simulink model "GHAME_Public"  (R2024a)
settings: Solver=ode8  StartTime=0.0  StopTime=Sim.simulation.duration  FixedStep=0.01  RelTol=1e-3
undefined symbols (not defined in the file): Data, DataPlant, IC, Sim, v0_BE_B
libraries: simulink_extras x8, simulink x1
(part 1 of 3)
settings Model: PacingRate=1000  Creator=Thoma  LastModifiedBy=muel_td
settings SolverCC: AlgebraicLoopSolver=TrustRegion  PositivePriorityOrder=on  MinimalZcImpactIntegration=on
settings DataIOCC: ExternalInput=getinputstruct(report2)  InitialState=getstatestruct(report2)
settings OptimizationCC: SimCompilerOptimization=on  AccelVerboseBuild=on
settings DebuggingCC: RTPrefix=none  StringTruncationChecking=none  ReadBeforeWriteMsg=DisableAll  WriteAfterWriteMsg=DisableAll  WriteAfterReadMsg=DisableAll  AlgebraicLoopMsg=none  SignalResolutionControl=None  MultiTaskDSMMsg=none  IntegerOverflowMsg=none  ParameterDowncastMsg=none  ParameterOverflowMsg=none  ParameterPrecisionLossMsg=none  ParameterTunabilityLossMsg=none  IntegerSaturationMsg=none  ArithmeticOperatorsInVariantConditions=warning
settings ModelReferenceCC: UpdateModelReferenceTargets=IfOutOfDate
settings SFSimCC: SFSimEcho=off  CustomCodeUndefinedFunction=UseInterfaceOnly
settings RTWCC: GPUComputeCapability=3.5

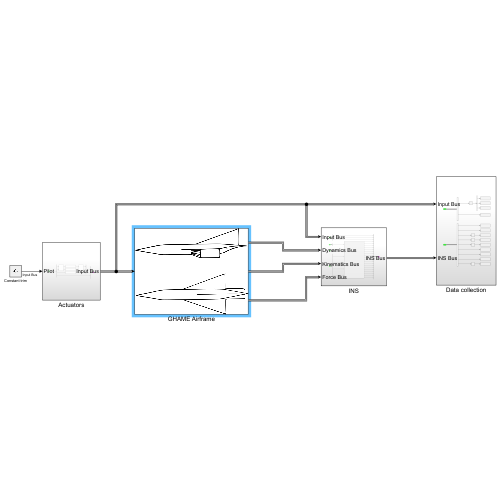
[thumbnail: Simulink's stored preview of the top-level diagram]
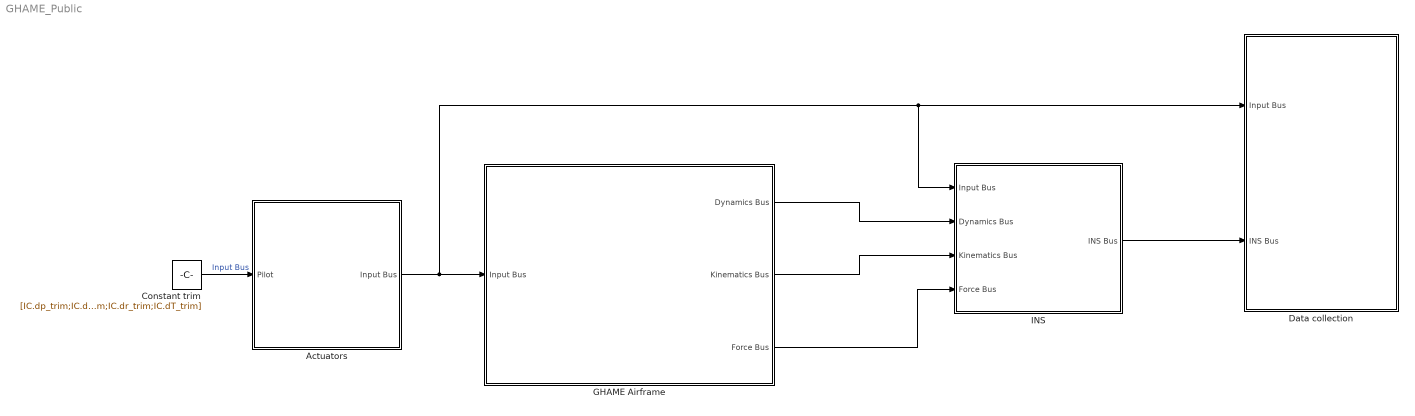
== system GHAME_Public ==
  Actuators : Subsystem
  Constant trim : Constant  Value=[IC.dp_trim;IC.dq_trim;IC.dr_trim;IC.dT_trim]
  Data collection : Subsystem
  GHAME Airframe : Subsystem
      mask Display: image('GHAME.png');
  INS : Subsystem
  wires:
  Actuators/1(Input Bus) -> GHAME Airframe/1(Input Bus), INS/1(Input Bus), Data collection/1(Input Bus)
  Constant trim/1 -> Actuators/1(Pilot)  "Input Bus"
  GHAME Airframe/2(Kinematics Bus) -> INS/3(Kinematics Bus)
  GHAME Airframe/1(Dynamics Bus) -> INS/2(Dynamics Bus)
  INS/1(INS Bus) -> Data collection/2(INS Bus)
  GHAME Airframe/3(Force Bus) -> INS/4(Force Bus)

== system GHAME_Public/Actuators ==
  Pilot : Inport
  Bus Creator : BusCreator  Inputs=2
  Demux : Demux
  Mux : Mux  Inputs=3
  Subsystem : Subsystem
  Subsystem1 : Subsystem
  Subsystem2 : Subsystem
  from Elevon command : Subsystem
  to Elevon command : Subsystem
  Input Bus : Outport
  wires:
  from Elevon command/1(dela) -> Mux/1  "Aileron"
  Demux/3 -> Subsystem2/1(delrc)
  to Elevon command/2(elvrc) -> Subsystem1/1(elvrc)
  Demux/1 -> to Elevon command/1(delac)
  to Elevon command/1(elvlc) -> Subsystem/1(elvlc)
  Demux/2 -> to Elevon command/2(delec)
  Subsystem/1(elvl) -> from Elevon command/1(elvl)
  Subsystem2/1(delr) -> Mux/3  "Rudder"
  Bus Creator/1 -> Input Bus/1
  Demux/4 -> Bus Creator/2  "thrtl"
  from Elevon command/2(dele) -> Mux/2  "Elevator"
  Mux/1 -> Bus Creator/1  "Deflections (rad)"
  Subsystem1/1(elvr) -> from Elevon command/2(elvr)
  Pilot/1 -> Demux/1

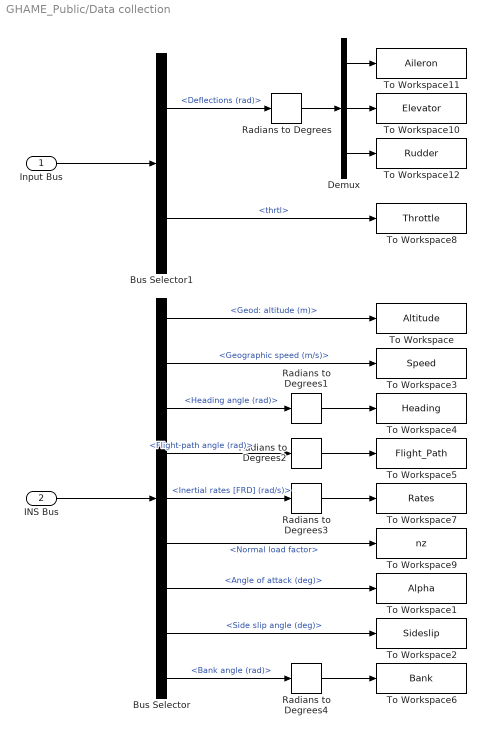
== system GHAME_Public/Data collection ==
  Input Bus : Inport
  INS Bus : Inport  Port=2
  Bus Selector : BusSelector  OutputSignals=Geod: altitude (m),Geographic speed (m/s),Heading angle (rad),Flight-path angle (rad),Inertial rates [FRD] (rad/s),Normal load factor,Angle of attack (deg),Side slip angle (deg),Bank angle (rad)
  Bus Selector1 : BusSelector  OutputSignals=Deflections (rad),thrtl
  Demux : Demux  Outputs=3
  Radians to Degrees{,1..4} (5 alike) : simulink_extras/Transformations/Radians to Degrees
  To Workspace : ToWorkspace  VariableName=Altitude  SampleTime=Sim.sample_time
  To Workspace1 : ToWorkspace  VariableName=Alpha  SampleTime=Sim.sample_time
  To Workspace10 : ToWorkspace  VariableName=Elevator  SampleTime=Sim.sample_time
  To Workspace11 : ToWorkspace  VariableName=Aileron  SampleTime=Sim.sample_time
  To Workspace12 : ToWorkspace  VariableName=Rudder  SampleTime=Sim.sample_time
  To Workspace2 : ToWorkspace  VariableName=Sideslip  SampleTime=Sim.sample_time
  To Workspace3 : ToWorkspace  VariableName=Speed  SampleTime=Sim.sample_time
  To Workspace4 : ToWorkspace  VariableName=Heading  SampleTime=Sim.sample_time
  To Workspace5 : ToWorkspace  VariableName=Flight_Path  SampleTime=Sim.sample_time
  To Workspace6 : ToWorkspace  VariableName=Bank  SampleTime=Sim.sample_time
  To Workspace7 : ToWorkspace  VariableName=Rates  SampleTime=Sim.sample_time
  To Workspace8 : ToWorkspace  VariableName=Throttle  SampleTime=Sim.sample_time
  To Workspace9 : ToWorkspace  VariableName=nz  SampleTime=Sim.sample_time
  wires:
  INS Bus/1 -> Bus Selector/1
  Bus Selector/1 -> To Workspace/1  "<Geod: altitude (m)>"
  Bus Selector/2 -> To Workspace3/1  "<Geographic speed (m/s)>"
  Bus Selector/3 -> Radians to Degrees1/1  "<Heading angle (rad)>"
  Bus Selector/4 -> Radians to Degrees2/1  "<Flight-path angle (rad)>"
  Bus Selector/5 -> Radians to Degrees3/1  "<Inertial rates [FRD] (rad/s)>"
  Bus Selector/6 -> To Workspace9/1  "<Normal load factor>"
  Bus Selector/7 -> To Workspace1/1  "<Angle of attack (deg)>"
  Bus Selector/8 -> To Workspace2/1  "<Side slip angle (deg)>"
  Bus Selector/9 -> Radians to Degrees4/1  "<Bank angle (rad)>"
  Input Bus/1 -> Bus Selector1/1
  Demux/1 -> To Workspace11/1
  Demux/2 -> To Workspace10/1
  Demux/3 -> To Workspace12/1
  Radians to Degrees1/1 -> To Workspace4/1
  Radians to Degrees2/1 -> To Workspace5/1
  Radians to Degrees3/1 -> To Workspace7/1
  Radians to Degrees4/1 -> To Workspace6/1
  Radians to Degrees/1 -> Demux/1
  Bus Selector1/2 -> To Workspace8/1  "<thrtl>"
  Bus Selector1/1 -> Radians to Degrees/1  "<Deflections (rad)>"

== system GHAME_Public/GHAME Airframe ==
  Input Bus : Inport
  Dynamics : Subsystem  Priority=4
  Environment : Subsystem  Priority=1
  Forces and Moments : Subsystem
  Kinematics : Subsystem  Priority=2
  Dynamics Bus : Outport
  Kinematics Bus : Outport  Port=2
  Force Bus : Outport  Port=3
  wires:
  Kinematics/1(Kinematics Bus) -> Forces and Moments/4(Kinematics Bus), Environment/2(Kinematics Bus), Kinematics Bus/1, Dynamics/3(Kinematics Bus)
  Dynamics/1(Dynamics Bus) -> Dynamics Bus/1, Forces and Moments/2(Dynamics Bus), Environment/1(Dynamics Bus), Kinematics/1(Dynamics Bus)
  Environment/1(Environment Bus) -> Forces and Moments/3(Environment Bus), Dynamics/2(Environment Bus)
  Forces and Moments/1(Force Bus) -> Dynamics/1(Force Bus), Force Bus/1
  Input Bus/1 -> Forces and Moments/1(Input Bus)

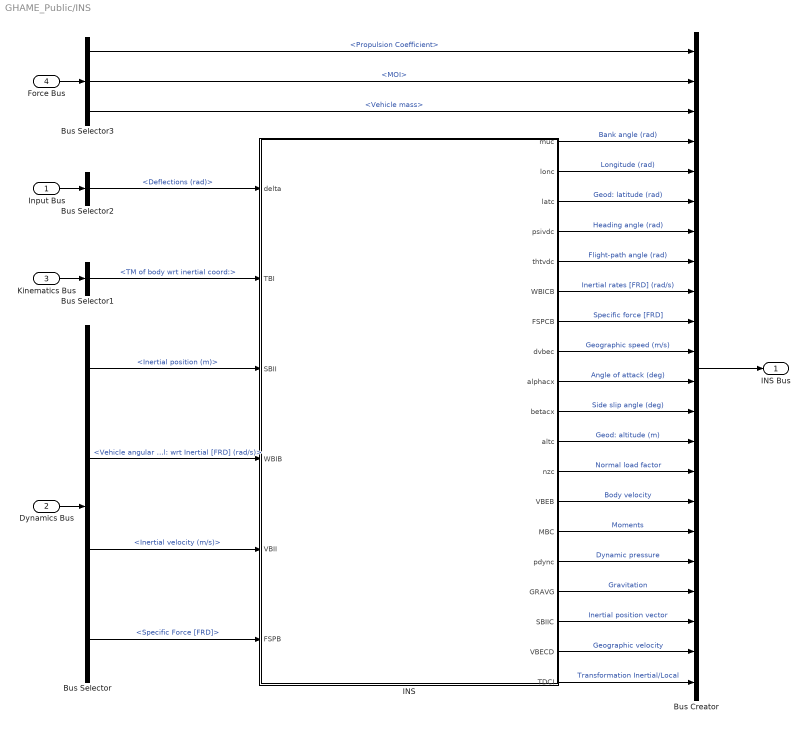
== system GHAME_Public/INS ==
  Input Bus : Inport
  Dynamics Bus : Inport  Port=2
  Kinematics Bus : Inport  Port=3
  Force Bus : Inport  Port=4
  Bus Creator : BusCreator  Inputs=22
  Bus Selector : BusSelector  OutputSignals=Newton Bus.Inertial position (m),Euler Bus.Vehicle angular vel: wrt Inertial [FRD] (rad/s),Newton Bus.Inertial velocity (m/s),Newton Bus.Specific Force [FRD]
  Bus Selector1 : BusSelector  OutputSignals=TM of body wrt inertial coord:
  Bus Selector2 : BusSelector  OutputSignals=Deflections (rad)
  Bus Selector3 : BusSelector  OutputSignals=Prop: data.Propulsion Coefficient,Prop: data.Mass and MOI.MOI,Prop: data.Mass and MOI.Vehicle mass
  INS : Subsystem
  INS Bus : Outport
  wires:
  INS/7(FSPCB) -> Bus Creator/10  "Specific force [FRD]"
  INS/5(thtvdc) -> Bus Creator/8  "Flight-path angle (rad)"
  INS/8(dvbec) -> Bus Creator/11  "Geographic speed (m/s)"
  INS/9(alphacx) -> Bus Creator/12  "Angle of attack (deg)"
  INS/6(WBICB) -> Bus Creator/9  "Inertial rates [FRD] (rad/s)"
  INS/4(psivdc) -> Bus Creator/7  "Heading angle (rad)"
  INS/10(betacx) -> Bus Creator/13  "Side slip angle (deg)"
  INS/1(muc) -> Bus Creator/4  "Bank angle (rad)"
  INS/2(lonc) -> Bus Creator/5  "Longitude (rad)"
  INS/11(altc) -> Bus Creator/14  "Geod: altitude (m)"
  INS/3(latc) -> Bus Creator/6  "Geod: latitude (rad)"
  Bus Selector/1 -> INS/3(SBII)  "<Inertial position (m)>"
  Bus Selector/3 -> INS/5(VBII)  "<Inertial velocity (m/s)>"
  Dynamics Bus/1 -> Bus Selector/1
  Bus Selector/2 -> INS/4(WBIB)  "<Vehicle angular vel: wrt Inertial [FRD] (rad/s)>"
  Bus Selector/4 -> INS/6(FSPB)  "<Specific Force [FRD]>"
  Kinematics Bus/1 -> Bus Selector1/1
  Bus Selector1/1 -> INS/2(TBI)  "<TM of body wrt inertial coord:>"
  Bus Creator/1 -> INS Bus/1
  INS/12(nzc) -> Bus Creator/15  "Normal load factor"
  INS/13(VBEB) -> Bus Creator/16  "Body velocity"
  Input Bus/1 -> Bus Selector2/1
  Bus Selector2/1 -> INS/1(delta)  "<Deflections (rad)>"
  Force Bus/1 -> Bus Selector3/1
  Bus Selector3/2 -> Bus Creator/2  "<MOI>"
  INS/14(MBC) -> Bus Creator/17  "Moments"
  INS/15(pdync) -> Bus Creator/18  "Dynamic pressure"
  Bus Selector3/3 -> Bus Creator/3  "<Vehicle mass>"
  INS/16(GRAVG) -> Bus Creator/19  "Gravitation"
  Bus Selector3/1 -> Bus Creator/1  "<Propulsion Coefficient>"
  INS/17(SBIIC) -> Bus Creator/20  "Inertial position vector"
  INS/18(VBECD) -> Bus Creator/21  "Geographic velocity"
  INS/19(TDCI) -> Bus Creator/22  "Transformation Inertial/Local"

== system GHAME_Public/Actuators/Subsystem ==
  elvlc : Inport
  2*zeta * wn : Gain  Gain=2*Sim.actuator.zeta*Sim.actuator.omega  SaturateOnIntegerOverflow=on  OutDataTypeStr=Inherit: Same as input  ParamDataTypeStr=Inherit: Same as input
  Demand limits : Saturate  UpperLimit=Sim.actuator.defl_lim_deg*Sim.constants.RAD  LowerLimit=-Sim.actuator.defl_lim_deg*Sim.constants.RAD
  "Integrator, Second-Order Limited" : SecondOrderIntegrator  ICX=IC.dp_trim+IC.dq_trim  LimitX=on  UpperLimitX=Sim.actuator.defl_lim_deg*Sim.constants.RAD  LowerLimitX=-Sim.actuator.defl_lim_deg*Sim.constants.RAD  ICDXDT=0  LimitDXDT=on  UpperLimitDXDT=Sim.actuator.rate_lim_deg*Sim.constants.RAD  LowerLimitDXDT=-Sim.actuator.rate_lim_deg*Sim.constants.RAD
  Sum2 : Sum  Inputs=|+-  InputSameDT=on  SaturateOnIntegerOverflow=on  OutDataTypeStr=Inherit: Same as first input
  Sum3 : Sum  Inputs=|+-  InputSameDT=on  SaturateOnIntegerOverflow=on  OutDataTypeStr=Inherit: Same as first input
  rate limit*2*zeta/wn : Saturate  UpperLimit=Sim.actuator.rate_lim_deg*2*Sim.actuator.zeta/Sim.actuator.omega*Sim.constants.RAD  LowerLimit=-Sim.actuator.rate_lim_deg*2*Sim.actuator.zeta/Sim.actuator.omega*Sim.constants.RAD
  wn^2 : Gain  Gain=Sim.actuator.omega^2  SaturateOnIntegerOverflow=on  OutDataTypeStr=Inherit: Same as input  ParamDataTypeStr=Inherit: Same as input
  elvl : Outport
  wires:
  wn^2/1 -> Sum2/1
  Sum3/1 -> rate limit*2*zeta/wn/1
  Sum2/1 -> "Integrator, Second-Order Limited"/1
  Demand limits/1 -> Sum3/1
  "Integrator, Second-Order Limited"/2 -> 2*zeta * wn/1
  "Integrator, Second-Order Limited"/1 -> Sum3/2, elvl/1
  2*zeta * wn/1 -> Sum2/2
  rate limit*2*zeta/wn/1 -> wn^2/1
  elvlc/1 -> Demand limits/1

== system GHAME_Public/Actuators/Subsystem1 ==
  elvrc : Inport
  2*zeta * wn : Gain  Gain=2*Sim.actuator.zeta*Sim.actuator.omega  SaturateOnIntegerOverflow=on  OutDataTypeStr=Inherit: Same as input  ParamDataTypeStr=Inherit: Same as input
  Demand limits : Saturate  UpperLimit=Sim.actuator.defl_lim_deg*Sim.constants.RAD  LowerLimit=-Sim.actuator.defl_lim_deg*Sim.constants.RAD
  "Integrator, Second-Order Limited" : SecondOrderIntegrator  ICX=IC.dq_trim-IC.dp_trim  LimitX=on  UpperLimitX=Sim.actuator.defl_lim_deg*Sim.constants.RAD  LowerLimitX=-Sim.actuator.defl_lim_deg*Sim.constants.RAD  ICDXDT=0  LimitDXDT=on  UpperLimitDXDT=Sim.actuator.rate_lim_deg*Sim.constants.RAD  LowerLimitDXDT=-Sim.actuator.rate_lim_deg*Sim.constants.RAD
  Sum2 : Sum  Inputs=|+-  InputSameDT=on  SaturateOnIntegerOverflow=on  OutDataTypeStr=Inherit: Same as first input
  Sum3 : Sum  Inputs=|+-  InputSameDT=on  SaturateOnIntegerOverflow=on  OutDataTypeStr=Inherit: Same as first input
  rate limit*2*zeta/wn : Saturate  UpperLimit=Sim.actuator.rate_lim_deg*2*Sim.actuator.zeta/Sim.actuator.omega*Sim.constants.RAD  LowerLimit=-Sim.actuator.rate_lim_deg*2*Sim.actuator.zeta/Sim.actuator.omega*Sim.constants.RAD
  wn^2 : Gain  Gain=Sim.actuator.omega^2  SaturateOnIntegerOverflow=on  OutDataTypeStr=Inherit: Same as input  ParamDataTypeStr=Inherit: Same as input
  elvr : Outport
  wires:
  2*zeta * wn/1 -> Sum2/2
  rate limit*2*zeta/wn/1 -> wn^2/1
  "Integrator, Second-Order Limited"/2 -> 2*zeta * wn/1
  wn^2/1 -> Sum2/1
  "Integrator, Second-Order Limited"/1 -> elvr/1, Sum3/2
  Demand limits/1 -> Sum3/1
  elvrc/1 -> Demand limits/1
  Sum2/1 -> "Integrator, Second-Order Limited"/1
  Sum3/1 -> rate limit*2*zeta/wn/1

== system GHAME_Public/Actuators/Subsystem2 ==
  delrc : Inport
  2*zeta * wn : Gain  Gain=2*Sim.actuator.zeta*Sim.actuator.omega  SaturateOnIntegerOverflow=on  OutDataTypeStr=Inherit: Same as input  ParamDataTypeStr=Inherit: Same as input
  Demand limits : Saturate  UpperLimit=Sim.actuator.defl_lim_deg*Sim.constants.RAD  LowerLimit=-Sim.actuator.defl_lim_deg*Sim.constants.RAD
  "Integrator, Second-Order Limited" : SecondOrderIntegrator  ICX=IC.dr_trim  LimitX=on  UpperLimitX=Sim.actuator.defl_lim_deg*Sim.constants.RAD  LowerLimitX=-Sim.actuator.defl_lim_deg*Sim.constants.RAD  ICDXDT=0  LimitDXDT=on  UpperLimitDXDT=Sim.actuator.rate_lim_deg*Sim.constants.RAD  LowerLimitDXDT=-Sim.actuator.rate_lim_deg*Sim.constants.RAD
  Sum2 : Sum  Inputs=|+-  InputSameDT=on  SaturateOnIntegerOverflow=on  OutDataTypeStr=Inherit: Same as first input
  Sum3 : Sum  Inputs=|+-  InputSameDT=on  SaturateOnIntegerOverflow=on  OutDataTypeStr=Inherit: Same as first input
  rate limit*2*zeta/wn : Saturate  UpperLimit=Sim.actuator.rate_lim_deg*2*Sim.actuator.zeta/Sim.actuator.omega*Sim.constants.RAD  LowerLimit=-Sim.actuator.rate_lim_deg*2*Sim.actuator.zeta/Sim.actuator.omega*Sim.constants.RAD
  wn^2 : Gain  Gain=Sim.actuator.omega^2  SaturateOnIntegerOverflow=on  OutDataTypeStr=Inherit: Same as input  ParamDataTypeStr=Inherit: Same as input
  delr : Outport
  wires:
  delrc/1 -> Demand limits/1
  Sum2/1 -> "Integrator, Second-Order Limited"/1
  Sum3/1 -> rate limit*2*zeta/wn/1
  "Integrator, Second-Order Limited"/2 -> 2*zeta * wn/1
  rate limit*2*zeta/wn/1 -> wn^2/1
  2*zeta * wn/1 -> Sum2/2
  wn^2/1 -> Sum2/1
  "Integrator, Second-Order Limited"/1 -> delr/1, Sum3/2
  Demand limits/1 -> Sum3/1

== system GHAME_Public/Actuators/from Elevon command ==
  elvl : Inport
  elvr : Inport  Port=2
  Add : Sum  Inputs=+-
  Add1 : Sum
  Constant : Constant  Value=2
  Divide : Product  Inputs=*/
  Divide1 : Product  Inputs=/*
  dela : Outport
  dele : Outport  Port=2
  wires:
  Add/1 -> Divide/1
  Add1/1 -> Divide1/2
  elvl/1 -> Add/1, Add1/2
  elvr/1 -> Add/2, Add1/1
  Divide/1 -> dela/1
  Constant/1 -> Divide1/1, Divide/2
  Divide1/1 -> dele/1

== system GHAME_Public/Actuators/to Elevon command ==
  delac : Inport
  delec : Inport  Port=2
  Add : Sum
  Add1 : Sum
  Unary Minus : UnaryMinus
  elvlc : Outport
  elvrc : Outport  Port=2
  wires:
  Add1/1 -> elvrc/1
  delac/1 -> Unary Minus/1, Add/1
  Unary Minus/1 -> Add1/2
  delec/1 -> Add1/1, Add/2
  Add/1 -> elvlc/1

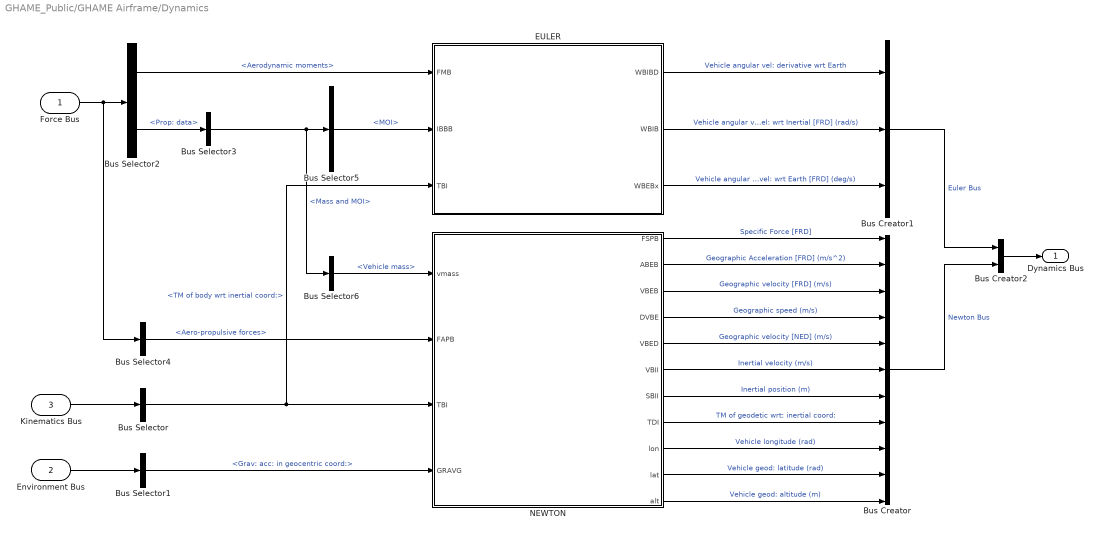
== system GHAME_Public/GHAME Airframe/Dynamics ==
  Force Bus : Inport
  Environment Bus : Inport  Port=2
  Kinematics Bus : Inport  Port=3
  Bus Creator : BusCreator  Inputs=11
  Bus Creator1 : BusCreator  Inputs=3
  Bus Creator2 : BusCreator  Inputs=2
  Bus Selector : BusSelector  OutputSignals=TM of body wrt inertial coord:
  Bus Selector1 : BusSelector  OutputSignals=Grav: acc: in geocentric coord:
  Bus Selector2 : BusSelector  OutputSignals=Aerodynamic moments,Prop: data
  Bus Selector3 : BusSelector  OutputSignals=Mass and MOI
  Bus Selector4 : BusSelector  OutputSignals=Aero-propulsive forces
  Bus Selector5 : BusSelector  OutputSignals=MOI
  Bus Selector6 : BusSelector  OutputSignals=Vehicle mass
  EULER : Subsystem
  NEWTON : Subsystem
  Dynamics Bus : Outport
  wires:
  Bus Creator/1 -> Bus Creator2/2  "Newton Bus"
  EULER/3(WBEBx) -> Bus Creator1/3  "Vehicle angular vel: wrt Earth [FRD] (deg/s)"
  Kinematics Bus/1 -> Bus Selector/1
  Bus Selector/1 -> EULER/3(TBI), NEWTON/3(TBI)  "<TM of body wrt inertial coord:>"
  Bus Selector1/1 -> NEWTON/4(GRAVG)  "<Grav: acc: in geocentric coord:>"
  EULER/2("WBIB ") -> Bus Creator1/2  "Vehicle angular vel: wrt Inertial [FRD] (rad/s)"
  Environment Bus/1 -> Bus Selector1/1
  Bus Creator1/1 -> Bus Creator2/1  "Euler Bus"
  Bus Creator2/1 -> Dynamics Bus/1
  NEWTON/7("SBII ") -> Bus Creator/7  "Inertial position (m)"
  NEWTON/9(lon) -> Bus Creator/9  "Vehicle longitude (rad)"
  NEWTON/10(lat) -> Bus Creator/10  "Vehicle geod: latitude (rad)"
  NEWTON/11(alt) -> Bus Creator/11  "Vehicle geod: altitude (m)"
  NEWTON/8(TDI) -> Bus Creator/8  "TM of geodetic wrt: inertial coord:"
  NEWTON/5(VBED) -> Bus Creator/5  "Geographic velocity [NED] (m/s)"
  NEWTON/2(ABEB) -> Bus Creator/2  "Geographic Acceleration [FRD] (m/s^2)"
  NEWTON/4(DVBE) -> Bus Creator/4  "Geographic speed (m/s)"
  Force Bus/1 -> Bus Selector2/1, Bus Selector4/1
  Bus Selector2/1 -> EULER/1(FMB)  "<Aerodynamic moments>"
  Bus Selector2/2 -> Bus Selector3/1  "<Prop: data>"
  Bus Selector4/1 -> NEWTON/2(FAPB)  "<Aero-propulsive forces>"
  NEWTON/1(FSPB) -> Bus Creator/1  "Specific Force [FRD]"
  NEWTON/6(VBII) -> Bus Creator/6  "Inertial velocity (m/s)"
  Bus Selector3/1 -> Bus Selector5/1, Bus Selector6/1  "<Mass and MOI>"
  Bus Selector5/1 -> EULER/2(IBBB)  "<MOI>"
  Bus Selector6/1 -> NEWTON/1(vmass)  "<Vehicle mass>"
  NEWTON/3(VBEB) -> Bus Creator/3  "Geographic velocity [FRD] (m/s)"
  EULER/1(WBIBD) -> Bus Creator1/1  "Vehicle angular vel: derivative wrt Earth"

== system GHAME_Public/GHAME Airframe/Environment ==
  Dynamics Bus : Inport
  Kinematics Bus : Inport  Port=2
  Bus Creator : BusCreator  Inputs=5
  Bus Selector : BusSelector  OutputSignals=Newton Bus.Inertial position (m),Newton Bus.Vehicle geod: altitude (m),Newton Bus.Vehicle geod: latitude (rad),Newton Bus.Vehicle longitude (rad),Newton Bus.Geographic velocity [NED] (m/s)
  Bus Selector1 : BusSelector  OutputSignals=Total angle of attack (deg),TM of body wrt geodetic coord:,Aeroballistic roll angle (deg)
  ENVIRONMENT : Subsystem  Priority=1
  Environment Bus : Outport
  wires:
  Dynamics Bus/1 -> Bus Selector/1
  Bus Creator/1 -> Environment Bus/1
  ENVIRONMENT/1(GRAVG) -> Bus Creator/1  "Grav: acc: in geocentric coord:"
  ENVIRONMENT/2(rho) -> Bus Creator/2  "Atmospheric density"
  ENVIRONMENT/3(pdynmc) -> Bus Creator/3  "Dynamic pressure"
  ENVIRONMENT/4(vmach) -> Bus Creator/4  "Mach number"
  ENVIRONMENT/5(DVBA) -> Bus Creator/5  "Speed of vehicle wrt air"
  Bus Selector/1 -> ENVIRONMENT/1(SBII)  "<Inertial position (m)>"
  Bus Selector/2 -> ENVIRONMENT/2(alt)  "<Vehicle geod: altitude (m)>"
  Bus Selector/5 -> ENVIRONMENT/5(VBED)  "<Geographic velocity [NED] (m/s)>"
  Bus Selector/4 -> ENVIRONMENT/4(lon)  "<Vehicle longitude (rad)>"
  Bus Selector/3 -> ENVIRONMENT/3(lat)  "<Vehicle geod: latitude (rad)>"
  Kinematics Bus/1 -> Bus Selector1/1
  Bus Selector1/2 -> ENVIRONMENT/7(TBD)  "<TM of body wrt geodetic coord:>"
  Bus Selector1/3 -> ENVIRONMENT/8(phipx)  "<Aeroballistic roll angle (deg)>"
  Bus Selector1/1 -> ENVIRONMENT/6(alppx)  "<Total angle of attack (deg)>"

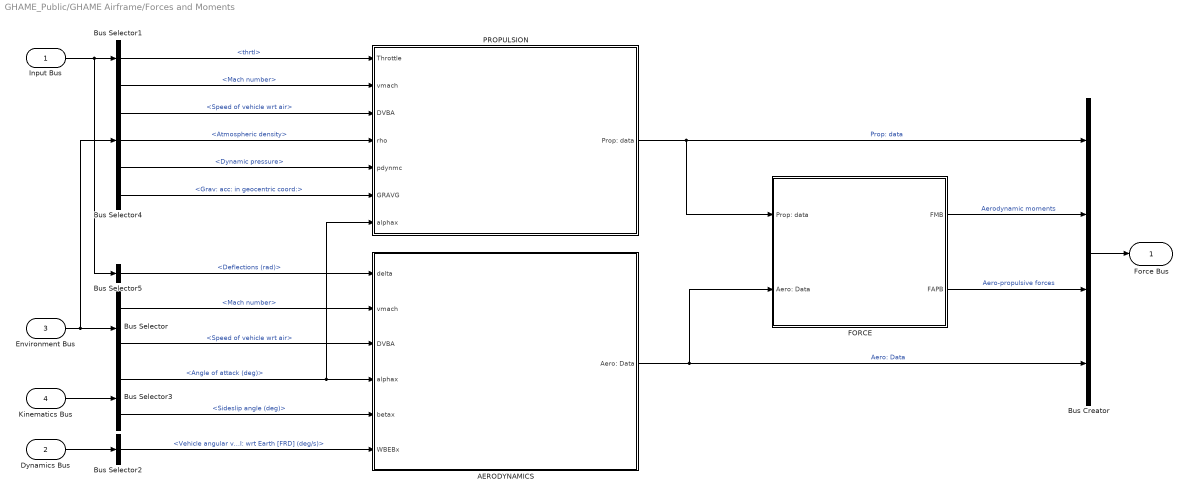
== system GHAME_Public/GHAME Airframe/Forces and Moments ==
  Input Bus : Inport  PortDimensions=4
  Dynamics Bus : Inport  Port=2
  Environment Bus : Inport  Port=3
  Kinematics Bus : Inport  Port=4
  AERODYNAMICS : Subsystem
  Bus Creator : BusCreator  Inputs=4
  Bus Selector : BusSelector  OutputSignals=Mach number,Speed of vehicle wrt air
  Bus Selector1 : BusSelector  OutputSignals=thrtl
  Bus Selector2 : BusSelector  OutputSignals=Euler Bus.Vehicle angular vel: wrt Earth [FRD] (deg/s)
  Bus Selector3 : BusSelector  OutputSignals=Angle of attack (deg),Sideslip angle (deg)
  Bus Selector4 : BusSelector  OutputSignals=Mach number,Speed of vehicle wrt air,Atmospheric density,Dynamic pressure,Grav: acc: in geocentric coord:
  Bus Selector5 : BusSelector  OutputSignals=Deflections (rad)
  FORCE : Subsystem
  PROPULSION : Subsystem
  Force Bus : Outport
  wires:
  FORCE/2(FAPB) -> Bus Creator/3  "Aero-propulsive forces"
  Environment Bus/1 -> Bus Selector4/1, Bus Selector/1
  Bus Selector/2 -> AERODYNAMICS/3(DVBA)  "<Speed of vehicle wrt air>"
  Dynamics Bus/1 -> Bus Selector2/1
  Kinematics Bus/1 -> Bus Selector3/1
  Input Bus/1 -> Bus Selector5/1, Bus Selector1/1
  Bus Selector3/1 -> AERODYNAMICS/4(alphax), PROPULSION/7(alphax)  "<Angle of attack (deg)>"
  Bus Selector4/4 -> PROPULSION/5(pdynmc)  "<Dynamic pressure>"
  FORCE/1(FMB) -> Bus Creator/2  "Aerodynamic moments"
  PROPULSION/1(Prop: data) -> FORCE/1(Prop: data), Bus Creator/1  "Prop: data"
  AERODYNAMICS/1(Aero: Data) -> FORCE/2(Aero: Data), Bus Creator/4  "Aero: Data"
  Bus Creator/1 -> Force Bus/1
  Bus Selector1/1 -> PROPULSION/1(Throttle)  "<thrtl>"
  Bus Selector/1 -> AERODYNAMICS/2(vmach)  "<Mach number>"
  Bus Selector4/3 -> PROPULSION/4(rho)  "<Atmospheric density>"
  Bus Selector3/2 -> AERODYNAMICS/5(betax)  "<Sideslip angle (deg)>"
  Bus Selector2/1 -> AERODYNAMICS/6(WBEBx)  "<Vehicle angular vel: wrt Earth [FRD] (deg/s)>"
  Bus Selector4/2 -> PROPULSION/3(DVBA)  "<Speed of vehicle wrt air>"
  Bus Selector4/1 -> PROPULSION/2(vmach)  "<Mach number>"
  Bus Selector4/5 -> PROPULSION/6(GRAVG)  "<Grav: acc: in geocentric coord:>"
  Bus Selector5/1 -> AERODYNAMICS/1(delta)  "<Deflections (rad)>"

== system GHAME_Public/GHAME Airframe/Kinematics ==
  Dynamics Bus : Inport
  Bus Creator : BusCreator  Inputs=7
  Bus Selector1 : BusSelector  OutputSignals=Euler Bus.Vehicle angular vel: wrt Inertial [FRD] (rad/s),Newton Bus.Geographic velocity [NED] (m/s),Newton Bus.TM of geodetic wrt: inertial coord:
  KINEMATICS : Subsystem
  Kinematics Bus : Outport
  wires:
  Bus Creator/1 -> Kinematics Bus/1
  Dynamics Bus/1 -> Bus Selector1/1
  KINEMATICS/3(alphax) -> Bus Creator/3  "Angle of attack (deg)"
  KINEMATICS/1("TBI ") -> Bus Creator/1  "TM of body wrt inertial coord:"
  KINEMATICS/2(TBD) -> Bus Creator/2  "TM of body wrt geodetic coord:"
  KINEMATICS/5(alppx) -> Bus Creator/5  "Total angle of attack (deg)"
  KINEMATICS/6(phipx) -> Bus Creator/6  "Aeroballistic roll angle (deg)"
  KINEMATICS/4(betax) -> Bus Creator/4  "Sideslip angle (deg)"
  Bus Selector1/1 -> KINEMATICS/1(WBIB)  "<Vehicle angular vel: wrt Inertial [FRD] (rad/s)>"
  KINEMATICS/7(phibdx) -> Bus Creator/7  "Body roll angle (deg)"
  Bus Selector1/2 -> KINEMATICS/2(VBED)  "<Geographic velocity [NED] (m/s)>"
  Bus Selector1/3 -> KINEMATICS/3(TDI)  "<TM of geodetic wrt: inertial coord:>"

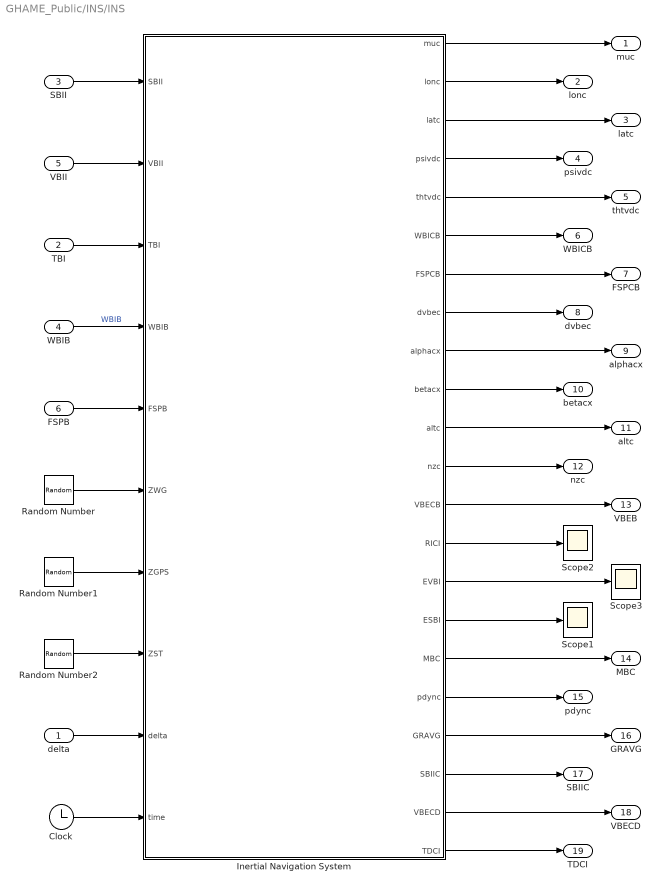
== system GHAME_Public/INS/INS ==
  delta : Inport
  TBI : Inport  Port=2
  SBII : Inport  Port=3
  WBIB : Inport  Port=4
  VBII : Inport  Port=5
  FSPB : Inport  Port=6
  Clock : Clock
  Inertial Navigation System : MATLAB Function  TreatAsAtomicUnit=on
  Random Number : RandomNumber  Seed=Sim.ins.seed_walk  SampleTime=Sim.sample_time
  Random Number1 : RandomNumber  Seed=Sim.gps.seed_noise  SampleTime=Sim.sample_time
  Random Number2 : RandomNumber  Seed=Sim.star.seed_noise  SampleTime=Sim.sample_time
  Scope1 : Scope
  Scope2 : Scope
  Scope3 : Scope
  muc : Outport
  lonc : Outport  Port=2
  latc : Outport  Port=3
  psivdc : Outport  Port=4
  thtvdc : Outport  Port=5
  WBICB : Outport  Port=6
  FSPCB : Outport  Port=7
  dvbec : Outport  Port=8
  alphacx : Outport  Port=9
  betacx : Outport  Port=10
  altc : Outport  Port=11
  nzc : Outport  Port=12
  VBEB : Outport  Port=13
  MBC : Outport  Port=14
  pdync : Outport  Port=15
  GRAVG : Outport  Port=16
  SBIIC : Outport  Port=17
  VBECD : Outport  Port=18
  TDCI : Outport  Port=19
  wires:
  SBII/1 -> Inertial Navigation System/1(SBII)
  VBII/1 -> Inertial Navigation System/2(VBII)
  TBI/1 -> Inertial Navigation System/3(TBI)
  Clock/1 -> Inertial Navigation System/10(time)
  WBIB/1 -> Inertial Navigation System/4(WBIB)  "WBIB"
  FSPB/1 -> Inertial Navigation System/5(FSPB)
  Inertial Navigation System/2(lonc) -> lonc/1
  Inertial Navigation System/12(nzc) -> nzc/1
  Inertial Navigation System/10(betacx) -> betacx/1
  Inertial Navigation System/9(alphacx) -> alphacx/1
  Inertial Navigation System/8(dvbec) -> dvbec/1
  Inertial Navigation System/7(FSPCB) -> FSPCB/1
  Inertial Navigation System/6(WBICB) -> WBICB/1
  Inertial Navigation System/1(muc) -> muc/1
  Inertial Navigation System/3(latc) -> latc/1
  Inertial Navigation System/4(psivdc) -> psivdc/1
  Inertial Navigation System/5(thtvdc) -> thtvdc/1
  Inertial Navigation System/13(VBECB) -> VBEB/1
  Random Number/1 -> Inertial Navigation System/6(ZWG)
  Random Number1/1 -> Inertial Navigation System/7(ZGPS)
  Inertial Navigation System/11(altc) -> altc/1
  Inertial Navigation System/16(ESBI) -> Scope1/1
  Inertial Navigation System/14(RICI) -> Scope2/1
  Random Number2/1 -> Inertial Navigation System/8(ZST)
  Inertial Navigation System/15(EVBI) -> Scope3/1
  delta/1 -> Inertial Navigation System/9(delta)
  Inertial Navigation System/17(MBC) -> MBC/1
  Inertial Navigation System/18(pdync) -> pdync/1
  Inertial Navigation System/19(GRAVG) -> GRAVG/1
  Inertial Navigation System/20(SBIIC) -> SBIIC/1
  Inertial Navigation System/21(VBECD) -> VBECD/1
  Inertial Navigation System/22(TDCI) -> TDCI/1

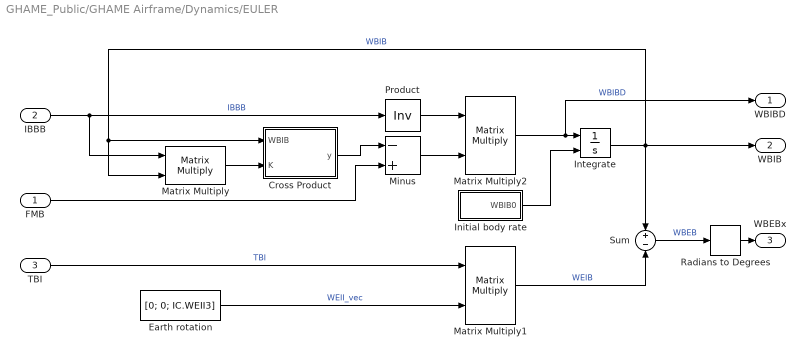
== system GHAME_Public/GHAME Airframe/Dynamics/EULER ==
  FMB : Inport
  IBBB : Inport  Port=2
  TBI : Inport  Port=3
  Cross Product : MATLAB Function  TreatAsAtomicUnit=on
  Earth rotation : Constant  Value=[0; 0; IC.WEII3]
  Initial body rate : Subsystem
  Integrate : Integrator  InitialConditionSource=external  InitialCondition=v0_BE_B
  Matrix Multiply : Product  Multiplication=Matrix(*)
  Matrix Multiply1 : Product  Multiplication=Matrix(*)
  Matrix Multiply2 : Product  Multiplication=Matrix(*)
  Minus : Sum  Inputs=-+
  Product : Product  Inputs=/  Multiplication=Matrix(*)  SaturateOnIntegerOverflow=on  OutDataTypeStr=Inherit: Same as first input
  Radians to Degrees : simulink_extras/Transformations/Radians to Degrees
  Sum : Sum  Inputs=+-
  WBIBD : Outport
  "WBIB " : Outport  Port=2
  WBEBx : Outport  Port=3
  wires:
  TBI/1 -> Matrix Multiply1/1  "TBI"
  Matrix Multiply1/1 -> Sum/2  "WEIB"
  FMB/1 -> Minus/2
  Matrix Multiply2/1 -> WBIBD/1, Integrate/1  "WBIBD"
  IBBB/1 -> Product/1, Matrix Multiply/1  "IBBB"
  Integrate/1 -> Sum/1, "WBIB "/1, Matrix Multiply/2, Cross Product/1(WBIB)  "WBIB"
  Earth rotation/1 -> Matrix Multiply1/2  "WEII_vec"
  Product/1 -> Matrix Multiply2/1
  Matrix Multiply/1 -> Cross Product/2(K)
  Cross Product/1(y) -> Minus/1
  Minus/1 -> Matrix Multiply2/2
  Radians to Degrees/1 -> WBEBx/1
  Sum/1 -> Radians to Degrees/1  "WBEB"
  Initial body rate/1(WBIB0) -> Integrate/2

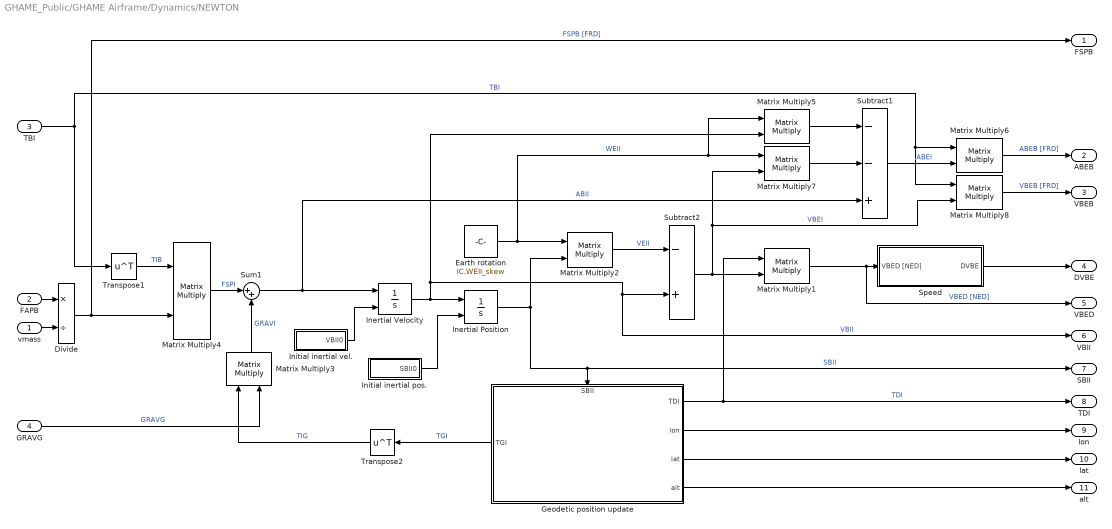
== system GHAME_Public/GHAME Airframe/Dynamics/NEWTON ==
  vmass : Inport
  FAPB : Inport  Port=2
  TBI : Inport  Port=3
  GRAVG : Inport  Port=4
  Divide : Product  Inputs=*/
  Earth rotation : Constant  Value=IC.WEII_skew
  Geodetic position update : Subsystem
      settings: PortSchema="{\"entries\":[{\"content\":{\"sides\":[{\"content\":{\"connectorIds\":[\"Out2\",\"Out3\",\"Out4\",\"Out5\"]},\"type\":\"ConnectorPlacement.EquallySpacedRectSide\",\"uuid\":\"7a13841f-bd3b-4040-beeb-525b1cd353ca\"},{\"content\":{\"connectorIds\":[\"Out1\"],\"side\":\"RIGHT\"},\"type\":\"ConnectorPlacement.EquallySpacedRectSide\",\"uuid\":\"57392278-0940-4a41-8639-f2af36fa41ab\"},{\"content\":{\"connectorIds\":[\"In1\"],\"side\":\"TOP\"},\"type\":\"ConnectorPlacement.EquallySpacedRectSide\",\"uuid\":\"d0e329d0-b4db-4dc4-8084-24bbc2802256\"}]},\"type\":\"ConnectorPlacement.EquallySpacedConnector\",\"uuid\":\"f3b20045-f33c-4e77-b986-a8c884bc766f\"}],\"packageUris\":[\"http://schema.mathworks.com/mf0/Connector/R2020b\"],\"version\":\"1.0\"}"
  Inertial Position : Integrator  InitialConditionSource=external  InitialCondition=IC.SBII
  Inertial Velocity : Integrator  InitialConditionSource=external  InitialCondition=v0_BE_B
  Initial inertial pos. : Subsystem
  Initial inertial vel. : Subsystem
  Matrix Multiply{1..8} (8 alike) : Product  Multiplication=Matrix(*)
  Speed : Subsystem
  Subtract1 : Sum  Inputs=--+
  Subtract2 : Sum  Inputs=-+
  Sum1 : Sum  Inputs=|++
  Transpose1 : Math  Operator=transpose  SignedPower=on
  Transpose2 : Math  Operator=transpose  SignedPower=on
  FSPB : Outport
  ABEB : Outport  Port=2
  VBEB : Outport  Port=3
  DVBE : Outport  Port=4
  VBED : Outport  Port=5
  VBII : Outport  Port=6
  "SBII " : Outport  Port=7
  TDI : Outport  Port=8
  lon : Outport  Port=9
  lat : Outport  Port=10
  alt : Outport  Port=11
  wires:
  Subtract2/1 -> Matrix Multiply1/2, Matrix Multiply8/2, Matrix Multiply7/2  "VBEI"
  Transpose1/1 -> Matrix Multiply4/1  "TIB"
  Inertial Position/1 -> Matrix Multiply2/2, Geodetic position update/1(SBII), "SBII "/1  "SBII"
  GRAVG/1 -> Matrix Multiply3/2  "GRAVG"
  Divide/1 -> Matrix Multiply4/2, FSPB/1  "FSPB [FRD]"
  Matrix Multiply4/1 -> Sum1/1  "FSPI"
  vmass/1 -> Divide/2
  Matrix Multiply2/1 -> Subtract2/1  "VEII"
  Matrix Multiply1/1 -> Speed/1(VBED [NED]), VBED/1  "VBED [NED]"
  FAPB/1 -> Divide/1
  Matrix Multiply3/1 -> Sum1/2  "GRAVI"
  Transpose2/1 -> Matrix Multiply3/1  "TIG"
  Geodetic position update/1(TGI) -> Transpose2/1  "TGI"
  Geodetic position update/5(alt) -> alt/1
  Geodetic position update/4(lat) -> lat/1
  Geodetic position update/3(lon) -> lon/1
  Geodetic position update/2(TDI) -> Matrix Multiply1/1, TDI/1  "TDI"
  Inertial Velocity/1 -> Inertial Position/1, Matrix Multiply5/2, VBII/1, Subtract2/2  "VBII"
  Sum1/1 -> Subtract1/3, Inertial Velocity/1  "ABII"
  Subtract1/1 -> Matrix Multiply6/2  "ABEI"
  Matrix Multiply5/1 -> Subtract1/1
  Earth rotation/1 -> Matrix Multiply2/1, Matrix Multiply7/1, Matrix Multiply5/1  "WEII"
  TBI/1 -> Matrix Multiply6/1, Matrix Multiply8/1, Transpose1/1  "TBI"
  Matrix Multiply6/1 -> ABEB/1  "ABEB [FRD]"
  Initial inertial vel./1(VBII0) -> Inertial Velocity/2
  Initial inertial pos./1(SBII0) -> Inertial Position/2
  Speed/1(DVBE) -> DVBE/1
  Matrix Multiply7/1 -> Subtract1/2
  Matrix Multiply8/1 -> VBEB/1  "VBEB [FRD]"

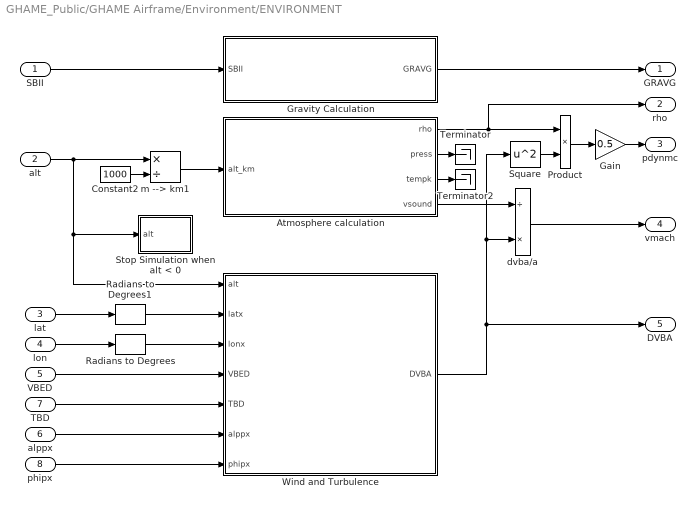
== system GHAME_Public/GHAME Airframe/Environment/ENVIRONMENT ==
  SBII : Inport
  alt : Inport  Port=2
  lat : Inport  Port=3
  lon : Inport  Port=4
  VBED : Inport  Port=5
  alppx : Inport  Port=6
  TBD : Inport  Port=7
  phipx : Inport  Port=8
  Atmosphere calculation : MATLAB Function  Priority=2  TreatAsAtomicUnit=on
  Constant2 : Constant  Value=1000
  Gain : Gain  Gain=0.5
  Gravity Calculation : MATLAB Function  Priority=1  TreatAsAtomicUnit=on
  Product : Product
  Radians to Degrees : simulink_extras/Transformations/Radians to Degrees
  Radians to Degrees1 : simulink_extras/Transformations/Radians to Degrees
  Square : Math  Operator=square  SignedPower=on
  Stop Simulation when alt < 0 : Subsystem
  Terminator : Terminator
  Terminator2 : Terminator
  Wind and Turbulence : Subsystem
  dvba/a : Product  Inputs=/*
  m --> km1 : Product  Inputs=*/
  GRAVG : Outport
  rho : Outport  Port=2
  pdynmc : Outport  Port=3
  vmach : Outport  Port=4
  DVBA : Outport  Port=5
  wires:
  SBII/1 -> Gravity Calculation/1(SBII)
  Constant2/1 -> m --> km1/2
  m --> km1/1 -> Atmosphere calculation/1(alt_km)
  Atmosphere calculation/4(vsound) -> dvba/a/1
  dvba/a/1 -> vmach/1
  Atmosphere calculation/1(rho) -> Product/1, rho/1
  Gravity Calculation/1(GRAVG) -> GRAVG/1
  Atmosphere calculation/3(tempk) -> Terminator2/1
  Atmosphere calculation/2(press) -> Terminator/1
  alt/1 -> Wind and Turbulence/1(alt), Stop Simulation when alt < 0/1(alt), m --> km1/1
  Wind and Turbulence/1(DVBA) -> DVBA/1, dvba/a/2, Square/1
  VBED/1 -> Wind and Turbulence/4(VBED)
  lat/1 -> Radians to Degrees1/1
  Radians to Degrees/1 -> Wind and Turbulence/3(lonx)
  Radians to Degrees1/1 -> Wind and Turbulence/2(latx)
  lon/1 -> Radians to Degrees/1
  Square/1 -> Product/2
  Product/1 -> Gain/1
  Gain/1 -> pdynmc/1
  TBD/1 -> Wind and Turbulence/5(TBD)
  alppx/1 -> Wind and Turbulence/6(alppx)
  phipx/1 -> Wind and Turbulence/7(phipx)

== system GHAME_Public/GHAME Airframe/Forces and Moments/AERODYNAMICS ==
  delta : Inport
  vmach : Inport  Port=2
  DVBA : Inport  Port=3
  alphax : Inport  Port=4
  betax : Inport  Port=5
  WBEBx : Inport  Port=6
  Aerodynamic Coefficients : MATLAB Function  TreatAsAtomicUnit=on
  Bus Creator2 : BusCreator  Inputs=2
  Aero: Data : Outport
  wires:
  vmach/1 -> Aerodynamic Coefficients/2(vmach)
  Aerodynamic Coefficients/2(c_moment) -> Bus Creator2/2  "Moment coefficients"
  DVBA/1 -> Aerodynamic Coefficients/3(DVBA)
  alphax/1 -> Aerodynamic Coefficients/4(alphax)
  Aerodynamic Coefficients/1(c_force) -> Bus Creator2/1  "Force coefficients"
  delta/1 -> Aerodynamic Coefficients/1(delta)
  Bus Creator2/1 -> Aero: Data/1
  WBEBx/1 -> Aerodynamic Coefficients/6(WBEBx)
  betax/1 -> Aerodynamic Coefficients/5(betax)

== system GHAME_Public/GHAME Airframe/Forces and Moments/FORCE ==
  Prop: data : Inport
  Aero: Data : Inport  Port=2
  Aerodynamic moments : MATLAB Function  TreatAsAtomicUnit=on
  Bus Selector : BusSelector  OutputSignals=Thrust,Dynamic pressure
  Bus Selector1 : BusSelector  OutputSignals=Force coefficients,Moment coefficients
  Non-gravitational forces : MATLAB Function  TreatAsAtomicUnit=on
  FMB : Outport
  FAPB : Outport  Port=2
  wires:
  Prop: data/1 -> Bus Selector/1
  Bus Selector/2 -> Non-gravitational forces/2(pdynmc), Aerodynamic moments/2(pdynmc)  "<Dynamic pressure>"
  Non-gravitational forces/1(FAPB) -> FAPB/1
  Bus Selector1/1 -> Non-gravitational forces/3(c_force)  "<Force coefficients>"
  Aerodynamic moments/1(FMB) -> FMB/1
  Bus Selector/1 -> Non-gravitational forces/1(Thrust)  "<Thrust>"
  Aero: Data/1 -> Bus Selector1/1
  Bus Selector1/2 -> Aerodynamic moments/1(c_moment)  "<Moment coefficients>"

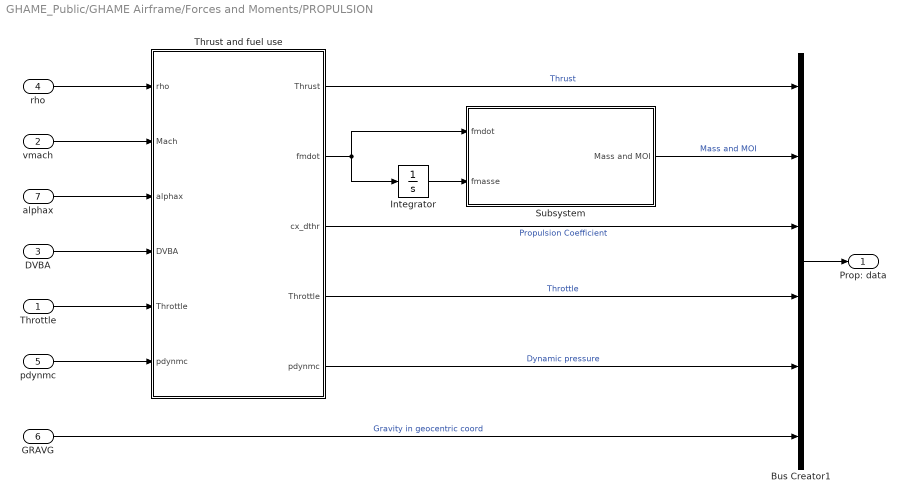
== system GHAME_Public/GHAME Airframe/Forces and Moments/PROPULSION ==
  Throttle : Inport  PortDimensions=1
  vmach : Inport  Port=2
  DVBA : Inport  Port=3
  rho : Inport  Port=4
  pdynmc : Inport  Port=5
  GRAVG : Inport  Port=6
  alphax : Inport  Port=7
  Bus Creator1 : BusCreator  Inputs=6
  Integrator : Integrator
  Subsystem : Subsystem
  Thrust and fuel use : MATLAB Function  TreatAsAtomicUnit=on
  Prop: data : Outport
  wires:
  alphax/1 -> Thrust and fuel use/3(alphax)
  Thrust and fuel use/2(fmdot) -> Integrator/1, Subsystem/1(fmdot)
  pdynmc/1 -> Thrust and fuel use/6("pdynmc ")
  vmach/1 -> Thrust and fuel use/2(Mach)
  rho/1 -> Thrust and fuel use/1(rho)
  DVBA/1 -> Thrust and fuel use/4(DVBA)
  Thrust and fuel use/1(Thrust) -> Bus Creator1/1  "Thrust"
  Throttle/1 -> Thrust and fuel use/5("Throttle ")
  Bus Creator1/1 -> Prop: data/1
  Thrust and fuel use/4(Throttle) -> Bus Creator1/4  "Throttle"
  GRAVG/1 -> Bus Creator1/6  "Gravity in geocentric coord"
  Integrator/1 -> Subsystem/2(fmasse)
  Subsystem/1(Mass and MOI) -> Bus Creator1/2  "Mass and MOI"
  Thrust and fuel use/3(cx_dthr) -> Bus Creator1/3  "Propulsion Coefficient"
  Thrust and fuel use/5(pdynmc) -> Bus Creator1/5  "Dynamic pressure"

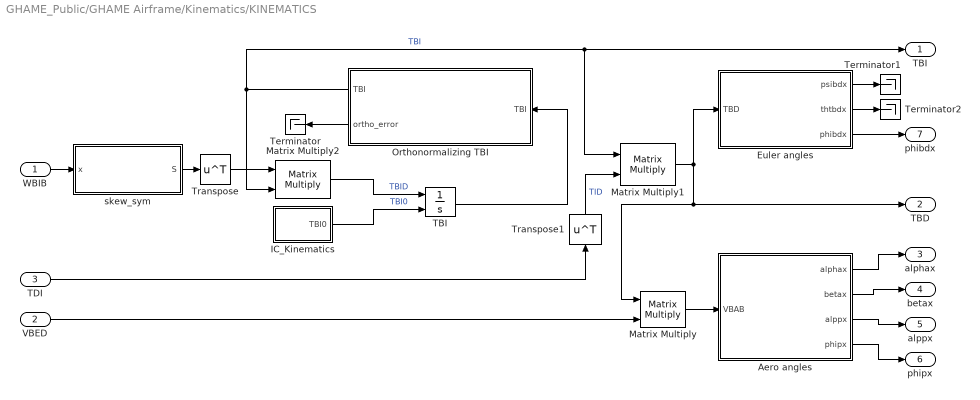
== system GHAME_Public/GHAME Airframe/Kinematics/KINEMATICS ==
  WBIB : Inport
  VBED : Inport  Port=2
  TDI : Inport  Port=3
  "\tOrthonormalizing TBI " : MATLAB Function  TreatAsAtomicUnit=on
  Aero angles : MATLAB Function  TreatAsAtomicUnit=on
  Euler angles : MATLAB Function  TreatAsAtomicUnit=on
  IC_Kinematics : Subsystem
  Matrix Multiply : Product  Multiplication=Matrix(*)
  Matrix Multiply1 : Product  Multiplication=Matrix(*)
  Matrix Multiply2 : Product  Multiplication=Matrix(*)
  "TBI  " : Integrator  InitialConditionSource=external  InitialCondition=v0_BE_B
  Terminator : Terminator
  Terminator1 : Terminator
  Terminator2 : Terminator
  Transpose : Math  Operator=transpose  SignedPower=on
  Transpose1 : Math  Operator=transpose  SignedPower=on
  skew_sym : MATLAB Function  TreatAsAtomicUnit=on
  "TBI " : Outport
  TBD : Outport  Port=2
  alphax : Outport  Port=3
  betax : Outport  Port=4
  alppx : Outport  Port=5
  phipx : Outport  Port=6
  phibdx : Outport  Port=7
  wires:
  WBIB/1 -> skew_sym/1(x)
  Euler angles/2(thtbdx) -> Terminator2/1
  TDI/1 -> Transpose1/1
  Euler angles/3(phibdx) -> phibdx/1
  "\tOrthonormalizing TBI "/1(TBI) -> Matrix Multiply2/2, "TBI "/1, Matrix Multiply1/1  "TBI"
  Matrix Multiply1/1 -> Euler angles/1(TBD), Matrix Multiply/1, TBD/1
  skew_sym/1(S) -> Transpose/1
  "\tOrthonormalizing TBI "/2(ortho_error) -> Terminator/1
  Transpose1/1 -> Matrix Multiply1/2  "TID"
  Euler angles/1(psibdx) -> Terminator1/1
  Transpose/1 -> Matrix Multiply2/1
  Matrix Multiply2/1 -> "TBI  "/1  "TBID"
  IC_Kinematics/1(TBI0) -> "TBI  "/2  "TBI0"
  "TBI  "/1 -> "\tOrthonormalizing TBI "/1("TBI ")
  VBED/1 -> Matrix Multiply/2
  Aero angles/1(alphax) -> alphax/1
  Aero angles/2(betax) -> betax/1
  Aero angles/3(alppx) -> alppx/1
  Aero angles/4(phipx) -> phipx/1
  Matrix Multiply/1 -> Aero angles/1(VBAB)

== system GHAME_Public/GHAME Airframe/Dynamics/EULER/Initial body rate ==
  Constant : Constant  Value=IC.WBIB
  WBIB0 : Outport
  wires:
  Constant/1 -> WBIB0/1

== system GHAME_Public/GHAME Airframe/Dynamics/NEWTON/Geodetic position update ==
  SBII : Inport
  Clock : Clock
  Geodetic Position : MATLAB Function  TreatAsAtomicUnit=on
  TM Inertial to Geocentric : MATLAB Function  TreatAsAtomicUnit=on
  TM Inertial to Geodetic : MATLAB Function  TreatAsAtomicUnit=on
  TGI : Outport
  TDI : Outport  Port=2
  lon : Outport  Port=3
  lat : Outport  Port=4
  alt : Outport  Port=5
  wires:
  SBII/1 -> Geodetic Position/2(SBII)
  Geodetic Position/1(lon) -> lon/1
  Geodetic Position/3(lat) -> TM Inertial to Geodetic/2("lat ")
  TM Inertial to Geodetic/1(TDI) -> TM Inertial to Geocentric/1("TDI ")
  Clock/1 -> Geodetic Position/1(time)
  TM Inertial to Geocentric/1(TGI) -> TGI/1
  Geodetic Position/2(lon_cel) -> TM Inertial to Geodetic/1(lon_cel)
  TM Inertial to Geocentric/4(alt) -> alt/1
  TM Inertial to Geocentric/3(lat) -> lat/1
  TM Inertial to Geocentric/2(TDI) -> TDI/1
  TM Inertial to Geodetic/2(lat) -> TM Inertial to Geocentric/2("lat ")
  Geodetic Position/4(alt) -> TM Inertial to Geocentric/3("alt ")

== system GHAME_Public/GHAME Airframe/Dynamics/NEWTON/Initial inertial pos. ==
  Constant : Constant  Value=IC.SBII
  SBII0 : Outport
  wires:
  Constant/1 -> SBII0/1

== system GHAME_Public/GHAME Airframe/Dynamics/NEWTON/Initial inertial vel. ==
  Constant : Constant  Value=IC.VBII
  VBII0 : Outport
  wires:
  Constant/1 -> VBII0/1

== system GHAME_Public/GHAME Airframe/Dynamics/NEWTON/Speed ==
  VBED [NED] : Inport
  Dot Product : DotProduct  OutDataTypeStr=Inherit: Inherit via internal rule
  Square Root : Sqrt
  DVBE : Outport
  wires:
  VBED [NED]/1 -> Dot Product/2, Dot Product/1
  Dot Product/1 -> Square Root/1
  Square Root/1 -> DVBE/1

== system GHAME_Public/GHAME Airframe/Environment/ENVIRONMENT/Stop Simulation when alt < 0 ==
  alt : Inport
  If : If  IfExpression=u1 <= 25  ShowElse=off
  Stop Simulationalt<0 : Subsystem  TreatAsAtomicUnit=on
  wires:
  If/1 -> Stop Simulationalt<0/Action
  alt/1 -> If/1

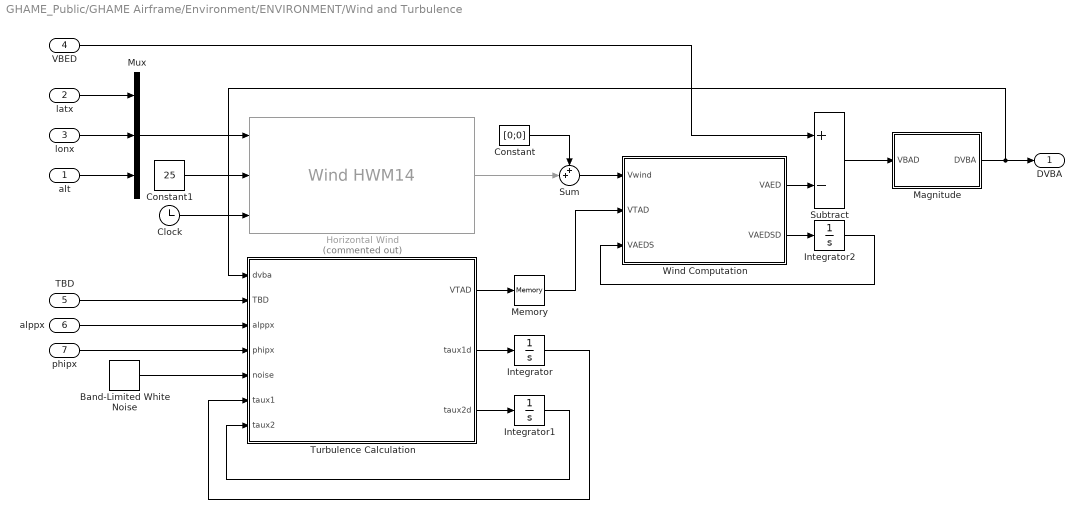
== system GHAME_Public/GHAME Airframe/Environment/ENVIRONMENT/Wind and Turbulence ==
  alt : Inport
  latx : Inport  Port=2
  lonx : Inport  Port=3
  VBED : Inport  Port=4
  TBD : Inport  Port=5
  alppx : Inport  Port=6
  phipx : Inport  Port=7
  Band-Limited White Noise : simulink/Sources/Band-Limited White Noise  Cov=1  Ts=Sim.sample_time  seed=Sim.uncertainty.seed
  Clock : Clock
  Constant : Constant  Value=[0;0]
  Constant1 : Constant  Value=25
  Horizontal Wind : WindHWM14  Commented=on
  Integrator : Integrator
  Integrator1 : Integrator
  Integrator2 : Integrator  InitialCondition=[0; 0; 0]
  Magnitude : MATLAB Function  TreatAsAtomicUnit=on
  Memory : Memory  InitialCondition=[0; 0; 0]
  Mux : Mux  Inputs=3
  Subtract : Sum  Inputs=+-
  Sum : Sum  Inputs=++|
  Turbulence Calculation : MATLAB Function  TreatAsAtomicUnit=on
  Wind Computation : MATLAB Function  TreatAsAtomicUnit=on
  DVBA : Outport
  wires:
  alt/1 -> Mux/3
  lonx/1 -> Mux/2
  Mux/1 -> Horizontal Wind/1
  Turbulence Calculation/2(taux1d) -> Integrator/1
  alppx/1 -> Turbulence Calculation/3(alppx)
  TBD/1 -> Turbulence Calculation/2(TBD)
  Clock/1 -> Horizontal Wind/3
  phipx/1 -> Turbulence Calculation/4(phipx)
  Constant1/1 -> Horizontal Wind/2
  Integrator2/1 -> Wind Computation/3(VAEDS)
  Subtract/1 -> Magnitude/1(VBAD)
  Integrator1/1 -> Turbulence Calculation/7(taux2)
  Integrator/1 -> Turbulence Calculation/6(taux1)
  Turbulence Calculation/3(taux2d) -> Integrator1/1
  latx/1 -> Mux/1
  VBED/1 -> Subtract/1
  Wind Computation/1(VAED) -> Subtract/2
  Wind Computation/2(VAEDSD) -> Integrator2/1
  Magnitude/1(DVBA) -> DVBA/1, Turbulence Calculation/1(dvba)
  Turbulence Calculation/1(VTAD) -> Memory/1
  Horizontal Wind/1 -> Sum/2
  Memory/1 -> Wind Computation/2(VTAD)
  Sum/1 -> Wind Computation/1(Vwind)
  Constant/1 -> Sum/1
  Band-Limited White Noise/1 -> Turbulence Calculation/5(noise)

== system GHAME_Public/GHAME Airframe/Forces and Moments/PROPULSION/Subsystem ==
  fmdot : Inport
  fmasse : Inport  Port=2
  Bus Creator : BusCreator  Inputs=3
  Stop Simulation : Stop
  Updating mass and inertia : MATLAB Function  TreatAsAtomicUnit=on
  Mass and MOI : Outport
  wires:
  Updating mass and inertia/3(vmass) -> Bus Creator/3  "Vehicle mass"
  Updating mass and inertia/4(stop_flag) -> Stop Simulation/1
  fmasse/1 -> Updating mass and inertia/2(fmasse)
  Updating mass and inertia/2(IBBBdot) -> Bus Creator/2  "MOI derivative"
  fmdot/1 -> Updating mass and inertia/1(fmdot)
  Updating mass and inertia/1(IBBB) -> Bus Creator/1  "MOI"
  Bus Creator/1 -> Mass and MOI/1

== system GHAME_Public/GHAME Airframe/Kinematics/KINEMATICS/IC_Kinematics ==
  Constant : Constant  Value=IC.TBI
  TBI0 : Outport
  wires:
  Constant/1 -> TBI0/1

== system GHAME_Public/GHAME Airframe/Environment/ENVIRONMENT/Stop Simulation when alt < 0/Stop Simulationalt<0 ==
  Action Port : ActionPort  ActionPortLabel=if(u1 <= 25)
  Constant2 : Constant
  Stop Simulation : Stop
  wires:
  Constant2/1 -> Stop Simulation/1

== matlab function GHAME_Public/GHAME Airframe/Forces and Moments/AERODYNAMICS/Aerodynamic Coefficients ==
  data: delta input; vmach input; DVBA input; c_force output double size=[3 1]; alphax input; betax input; WBEBx input; c_moment output double size=[3 1]; DataPlant parameter; Sim parameter
function [c_force, c_moment] = aerodynamics(delta, vmach, DVBA, alphax, betax, WBEBx, DataPlant, Sim)
% AERODYNAMICS  Aerodynamic force and moment coefficients of the GHAME
%   vehicle from the tabulated aero database.
%
%   [c_force, c_moment] = aerodynamics(delta, vmach, DVBA, alphax, betax, ...
%       WBEBx, Data, Sim)
%
%   Used in the plant. For Monte Carlo runs pass UNC.Perturbed from
%   Create_Uncertainty as Data, otherwise the nominal Data. The tables are
%   interpolated bilinearly in Mach and alpha, clamped to the table range.
%
%   Inputs
%     delta   [3x1]  Control surface deflections [aileron, elevator, rudder] (rad)
%     vmach   [1x1]  Mach number
%     DVBA    [1x1]  Airspeed (m/s)
%     alphax  [1x1]  Angle of attack (deg)
%     betax   [1x1]  Sideslip angle (deg)
%     WBEBx   [3x1]  Body rates [p, q, r] (deg/s)
%     Data    struct Aero tables and breakpoints (Data.AeroCoefficients)
%     Sim     struct Constants and vehicle geometry
%
%   Outputs
%     c_force   [3x1]  Body-axis force coefficients [Cx, Cy, Cz]
%     c_moment  [3x1]  Body-axis moment coefficients [Cl, Cm, Cn]
%
%   All table derivatives are per degree.

%   Author:    Thomas Harald Müller
%   GitHub:    https://github.com/ThomasHaraldMueller
%   Copyright: (c) 2026 Thomas Harald Müller, Hamburg, Germany
%   Free to use and modify, provided this notice is kept and the author is credited.

%% Constants and geometry
RAD  = Sim.constants.RAD;
DEG  = Sim.constants.DEG;
refb = Sim.vehicle.geometry.refb;
refc = Sim.vehicle.geometry.refc;

% Deflections in table units (deg)
delax = delta(1) * DEG;
delex = delta(2) * DEG;
delrx = delta(3) * DEG;

ppx = WBEBx(1);
qqx = WBEBx(2);
rrx = WBEBx(3);

%% Table lookup
Aero      = DataPlant.AeroCoefficients;
alpha_vec = Aero.alpha_vec;             % Breakpoints from the database (deg)
mach_vec  = Aero.Mach_vec;

vmach_c  = clamp_value(vmach,  mach_vec(1),  mach_vec(end));
alphax_c = clamp_value(alphax, alpha_vec(1), alpha_vec(end));

interp_coeff = @(table) interp2(mach_vec, alpha_vec, table, vmach_c, alphax_c, 'linear');

%% Stability-axis force coefficients
% Drag
cd0 = interp_coeff(Aero.CD0_tab);
cda = interp_coeff(Aero.CDA_tab);
cd  = cd0 + cda * alphax;

% Lift
cl0  = interp_coeff(Aero.CL0_tab);
cla  = interp_coeff(Aero.CLA_tab);
clde = interp_coeff(Aero.CLDE_tab);
cl   = cl0 + cla * alphax + clde * delex;

% Side force
cyb  = interp_coeff(Aero.CYB_tab);
cyda = interp_coeff(Aero.CYDA_tab);
cydr = interp_coeff(Aero.CYDR_tab);
cy   = cyb * betax + cyda * delax + cydr * delrx;

%% Body-axis moment coefficients
% Rate damping terms use the nondimensional rates p*b/(2V), q*c/(2V), r*b/(2V)
pn = ppx * RAD * refb / (2 * DVBA);
qn = qqx * RAD * refc / (2 * DVBA);
rn = rrx * RAD * refb / (2 * DVBA);

% Rolling moment
cllb  = interp_coeff(Aero.CLLB_tab);
cllda = interp_coeff(Aero.CLLDA_tab);
clldr = interp_coeff(Aero.CLLDR_tab);
cllp  = interp_coeff(Aero.CLLP_tab);
cllr  = interp_coeff(Aero.CLLR_tab);
cll   = cllb * betax + cllda * delax + clldr * delrx + cllp * pn + cllr * rn;

% Pitching moment
cm0  = interp_coeff(Aero.CM0_tab);
cma  = interp_coeff(Aero.CMA_tab);
cmde = interp_coeff(Aero.CMDE_tab);
cmq  = interp_coeff(Aero.CMQ_tab);
clm  = cm0 + cma * alphax + cmde * delex + cmq * qn;

% Yawing moment
clnb  = interp_coeff(Aero.CNB_tab);
clnda = interp_coeff(Aero.CNDA_tab);
clndr = interp_coeff(Aero.CNDR_tab);
clnp  = interp_coeff(Aero.CNP_tab);
clnr  = interp_coeff(Aero.CNR_tab);
cln   = clnb * betax + clnda * delax + clndr * delrx + clnp * pn + clnr * rn;

%% Body-axis outputs
% Rotation from stability axes (CD, CL) to body axes (Cx, Cz)
a  = alphax * RAD;
Cx = -cd * cos(a) + cl * sin(a);
Cz = -cd * sin(a) - cl * cos(a);

c_force  = [Cx; cy; Cz];
c_moment = [cll; clm; cln];

end

%% Local functions

function value_clamped = clamp_value(value, min_value, max_value)
% CLAMP_VALUE  Saturate value to [min_value, max_value]
    value_clamped = max(min(value, max_value), min_value);
end

== matlab function GHAME_Public/GHAME Airframe/Environment/ENVIRONMENT/Wind and Turbulence/Magnitude ==
  data: VBAD input; DVBA output
function DVBA = fcn(VBAD)
% Calculates magnitude of vector

DVBA = sqrt(VBAD(1)^2+VBAD(2)^2+VBAD(3)^2);

== matlab function GHAME_Public/GHAME Airframe/Dynamics/EULER/Cross Product ==
  data: WBIB input; y output; K input
function y = fcn(WBIB, K)


X=[0   -WBIB(3)   WBIB(2) ;
 WBIB(3)    0  -WBIB(1) ;
-WBIB(2)    WBIB(1)   0  ];

y = X*K;

== matlab function GHAME_Public/GHAME Airframe/Forces and Moments/FORCE/Non-gravitational forces ==
  data: Thrust input; pdynmc input; c_force input; FAPB output size=[3 1]; Sim parameter
function FAPB = computeForces(Thrust, pdynmc, c_force, Sim)
% COMPUTEFORCES  Aerodynamic and propulsive force in body axes.
%
%   FAPB = computeForces(Thrust, pdynmc, c_force, Sim)
%
%   Gravity is not included. Thrust is assumed to act along the body x-axis.
%
%   Inputs
%     Thrust   [1x1]  Thrust (N)
%     pdynmc   [1x1]  Dynamic pressure (Pa)
%     c_force  [3x1]  Body-axis force coefficients [Cx, Cy, Cz]
%     Sim      struct Vehicle geometry
%
%   Output
%     FAPB     [3x1]  Non-gravitational force in body axes [Fx, Fy, Fz] (N)

refa = Sim.vehicle.geometry.refa;
qS   = pdynmc * refa;

FAPB = qS * c_force(:) + [Thrust; 0; 0];

end

== matlab function GHAME_Public/GHAME Airframe/Environment/ENVIRONMENT/Wind and Turbulence/Turbulence Calculation ==
  settings: updateMethod=DISCRETE
  data: dvba input; TBD input; alppx input; phipx input; noise input; taux1 input; taux2 input; VTAD output; taux1d output; taux2d output; Sim parameter
function [VTAD, taux1d, taux2d] = environment_dryden(dvba, TBD, alppx, phipx, noise, taux1, taux2, Sim)
% ENVIRONMENT_DRYDEN  Dryden turbulence normal to the velocity vector.
%
%   [VTAD, taux1d, taux2d] = environment_dryden(TBD, alppx, phipx, dvba, ...
%       taux1, taux2, noise, Sim)
%
%   Second-order Dryden filter driven by unit white noise. The gust acts
%   perpendicular to the velocity in the load factor plane (normal gust only,
%   no longitudinal or lateral components). Transfer function
%
%     tau/noise = sigma*sqrt(L/(pi*V)) * (1 + sqrt(3)*(L/V)*s) / (1 + (L/V)*s)^2
%
%   Inputs
%     TBD      [3x3]  Transformation matrix, geodetic to body
%     alppx    [1x1]  Total angle of attack (deg)
%     phipx    [1x1]  Aerodynamic roll angle (deg)
%     dvba     [1x1]  Airspeed (m/s)
%     taux1    [1x1]  Filter state 1
%     taux2    [1x1]  Filter state 2
%     noise    [1x1]  White noise from a Band-Limited White Noise block with
%                     noise power 1 and sample time Sim.sample_time
%     Sim      struct Turbulence intensity and scale length
%
%   Outputs
%     VTAD     [3x1]  Turbulence velocity in geodetic axes (m/s)
%     taux1d   [1x1]  Derivative of filter state 1
%     taux2d   [1x1]  Derivative of filter state 2

%   Author:    Thomas Harald Müller
%   GitHub:    https://github.com/ThomasHaraldMueller
%   Copyright: (c) 2026 Thomas Harald Müller, Hamburg, Germany
%   Free to use and modify, provided this notice is kept and the author is credited.

RAD   = Sim.constants.RAD;
sigma = Sim.wind.turb_sigma;
L     = Sim.wind.turb_length;

% Inverse time constant V/L, protected against zero airspeed
vl = max(dvba, 1) / L;

% Filter states, denominator (s + vl)^2
taux1d = taux2;
taux2d = -vl^2 * taux1 - 2 * vl * taux2 + vl^2 * noise;

% Filter output, numerator 1 + sqrt(3)*s/vl
tau = sigma * sqrt(1 / (vl * pi)) * (taux1 + sqrt(3) * taux2 / vl);

% Unit vector normal to the velocity in the load factor plane
a = alppx * RAD;
p = phipx * RAD;
VTAB = tau * [-sin(a); sin(p) * cos(a); cos(p) * cos(a)];

VTAD = TBD * VTAB;

end
